simulink model "alveo_onehundred_gbe"  (R2021a)
settings: Solver=VariableStepAuto  StartTime=0.0  StopTime=10.0  RelTol=1e-3
libraries: xbsIndex_r4 x30
settings Model: Creator=qwerty40  LastModifiedBy=wnew
settings SolverCC: AlgebraicLoopSolver=TrustRegion
settings DataIOCC: ReturnWorkspaceOutputs=off
settings DebuggingCC: SFMachineParentedDataDiag=warning  ArithmeticOperatorsInVariantConditions=warning
settings SFSimCC: SimUseLocalCustomCode=off  CustomCodeUndefinedFunction=UseInterfaceOnly
settings RTWCC: RTWUseLocalCustomCode=off
settings CodeAppCC: StateflowObjectComments=on

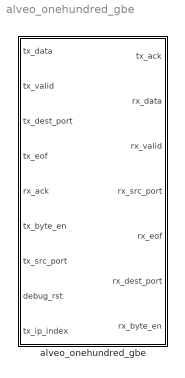
== system alveo_onehundred_gbe ==
  alveo_onehundred_gbe : Subsystem  Tag=xps:onehundred_gbe  mask(alveo_onehundred_gbe){Parameter1=off, fab_mac=hex2dec('123456780000'), fab_ip=192*(2^24) + 168*(2^16) + 5*(2^8) + 20*(2^0), fab_udp=10000}
      mask prompts: Parameter1 "Farm Mode"; fab_mac "Fabric MAC Address"; fab_ip "Fabric IP Address"; fab_udp "Fabric UDP Port"
      mask help: This block sends and receives UDP frames (packets). It accepts a 64 bit wide data stream with user-determined frame breaks. The data stream is wrapped in a UDP frame for transmission. Incoming UDP packets are unwrapped and the data presented as a 64 bit wide stream.
      mask init:
      | alveo_onehundred_gbe_mask(gcb)
      settings: AttributesFormatString=incoming_latency=0

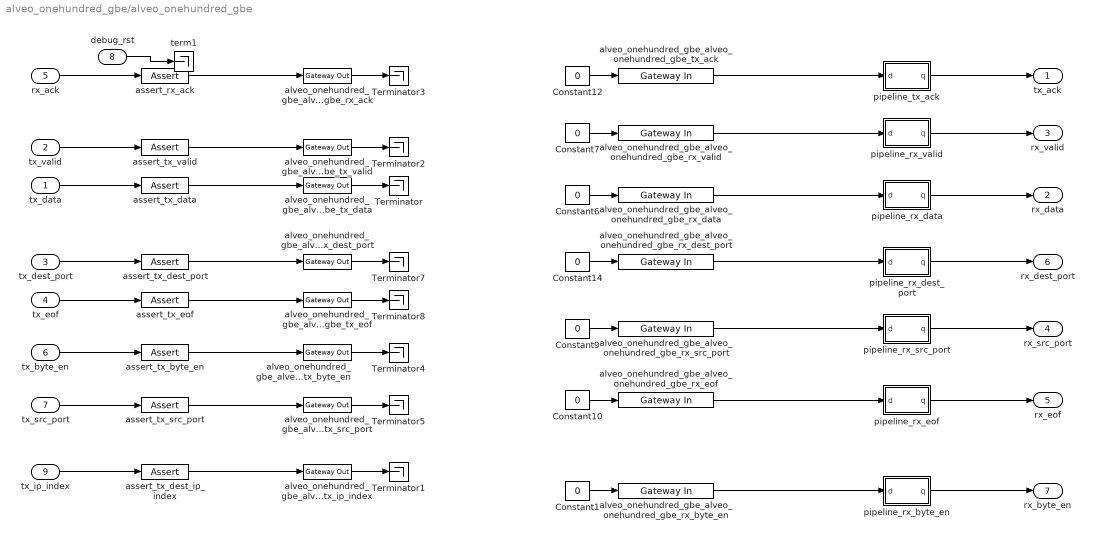
== system alveo_onehundred_gbe/alveo_onehundred_gbe ==
  tx_data : Inport
  tx_valid : Inport  Port=2
  tx_dest_port : Inport  Port=3
  tx_eof : Inport  Port=4
  rx_ack : Inport  Port=5
  tx_byte_en : Inport  Port=6
  tx_src_port : Inport  Port=7
  debug_rst : Inport  Port=8
  tx_ip_index : Inport  Port=9
  Constant{1,6..7,9..10,12,14} (7 alike) : Constant  Value=0
  Terminator{,1..5,7..8} (8 alike) : Terminator
  alveo_onehundred_gbe_alveo_onehundred_gbe_rx_ack : xbsIndex_r4/Gateway Out  inherit_from_input=off  hdl_port=on  rows=1  columns=1  UseAsDAC=off  DACChannel='1'  interface=None  automatic_assignment=on  address_offset=hex2dec('00')  intf_name=''  intf_description=''  timing_constraint=None  locs_specified=off  LOCs={}  io_standard={}  block_type=gatewayout
      settings: infoedit="Gateway out block.  Converts Xilinx fixed point inputs into ouputs of type Simulink integer, double, or fixed point.<P><P>Hardware notes:  In hardware these blocks become top level output ports or are discarded, depending on how they are configured."  xl_area=[0, 0, 0, 0, 0, 0, 0]
  alveo_onehundred_gbe_alveo_onehundred_gbe_rx_byte_en : xbsIndex_r4/Gateway In  gui_display_data_type=Fixed-point  arith_type=Unsigned  n_bits=64  bin_pt=0  preci_type=Single  exp_width=8  frac_width=24  rows=1  columns=1  quantization=Truncate  overflow=Wrap  period=1  UseAsADC=off  ADCChannel='1'  interface=None  automatic_assignment=on  address_offset=hex2dec('00')  intf_name=''  intf_description=''  default_value=0  timing_constraint=None  locs_specified=off  LOCs={}  io_standard={}  inherit_from_input=off  hdl_port=on  dbl_ovrd=off  block_type=gatewayin
      settings: xl_area=[0, 0, 0, 0, 0, 0, 0]
  alveo_onehundred_gbe_alveo_onehundred_gbe_rx_data : xbsIndex_r4/Gateway In  gui_display_data_type=Fixed-point  arith_type=Unsigned  n_bits=512  bin_pt=0  preci_type=Single  exp_width=8  frac_width=24  rows=1  columns=1  quantization=Truncate  overflow=Wrap  period=1  UseAsADC=off  ADCChannel='1'  interface=None  automatic_assignment=on  address_offset=hex2dec('00')  intf_name=''  intf_description=''  default_value=0  timing_constraint=None  locs_specified=off  LOCs={}  io_standard={}  inherit_from_input=off  hdl_port=on  dbl_ovrd=off  block_type=gatewayin
      settings: xl_area=[0, 0, 0, 0, 0, 0, 0]
  alveo_onehundred_gbe_alveo_onehundred_gbe_rx_dest_port : xbsIndex_r4/Gateway In  gui_display_data_type=Fixed-point  arith_type=Unsigned  n_bits=16  bin_pt=0  preci_type=Single  exp_width=8  frac_width=24  rows=1  columns=1  quantization=Truncate  overflow=Wrap  period=1  UseAsADC=off  ADCChannel='1'  interface=None  automatic_assignment=on  address_offset=hex2dec('00')  intf_name=''  intf_description=''  default_value=0  timing_constraint=None  locs_specified=off  LOCs={}  io_standard={}  inherit_from_input=off  hdl_port=on  dbl_ovrd=off  block_type=gatewayin
      settings: infoedit="Gateway in block.  Converts inputs of type Simulink integer, double and fixed point to  Xilinx fixed point type.<P><P>Hardware notes:  In hardware these blocks become top level input ports."  xl_area=[0, 0, 0, 0, 0, 0, 0]
  alveo_onehundred_gbe_alveo_onehundred_gbe_rx_eof : xbsIndex_r4/Gateway In  gui_display_data_type=Fixed-point  arith_type=Boolean  n_bits=1  bin_pt=0  preci_type=Single  exp_width=8  frac_width=24  rows=1  columns=1  quantization=Truncate  overflow=Wrap  period=1  UseAsADC=off  ADCChannel='1'  interface=None  automatic_assignment=on  address_offset=hex2dec('00')  intf_name=''  intf_description=''  default_value=0  timing_constraint=None  locs_specified=off  LOCs={}  io_standard={}  inherit_from_input=off  hdl_port=on  dbl_ovrd=off  block_type=gatewayin
      settings: infoedit="Gateway in block.  Converts inputs of type Simulink integer, double and fixed point to  Xilinx fixed point type.<P><P>Hardware notes:  In hardware these blocks become top level input ports."  xl_area=[0, 0, 0, 0, 0, 0, 0]
  alveo_onehundred_gbe_alveo_onehundred_gbe_rx_src_port : xbsIndex_r4/Gateway In  gui_display_data_type=Fixed-point  arith_type=Unsigned  n_bits=16  bin_pt=0  preci_type=Single  exp_width=8  frac_width=24  rows=1  columns=1  quantization=Truncate  overflow=Wrap  period=1  UseAsADC=off  ADCChannel='1'  interface=None  automatic_assignment=on  address_offset=hex2dec('00')  intf_name=''  intf_description=''  default_value=0  timing_constraint=None  locs_specified=off  LOCs={}  io_standard={}  inherit_from_input=off  hdl_port=on  dbl_ovrd=off  block_type=gatewayin
      settings: infoedit="Gateway in block.  Converts inputs of type Simulink integer, double and fixed point to  Xilinx fixed point type.<P><P>Hardware notes:  In hardware these blocks become top level input ports."  xl_area=[0, 0, 0, 0, 0, 0, 0]
  alveo_onehundred_gbe_alveo_onehundred_gbe_rx_valid : xbsIndex_r4/Gateway In  gui_display_data_type=Boolean  arith_type=Boolean  n_bits=4  bin_pt=0  preci_type=Single  exp_width=8  frac_width=24  rows=1  columns=1  quantization=Truncate  overflow=Wrap  period=1  UseAsADC=off  ADCChannel='1'  interface=None  automatic_assignment=on  address_offset=hex2dec('00')  intf_name=''  intf_description=''  default_value=0  timing_constraint=None  locs_specified=off  LOCs={}  io_standard={}  inherit_from_input=off  hdl_port=on  dbl_ovrd=off  block_type=gatewayin
      settings: xl_area=[0, 0, 0, 0, 0, 0, 0]
  alveo_onehundred_gbe_alveo_onehundred_gbe_tx_ack : xbsIndex_r4/Gateway In  gui_display_data_type=Boolean  arith_type=Boolean  n_bits=1  bin_pt=0  preci_type=Single  exp_width=8  frac_width=24  rows=1  columns=1  quantization=Truncate  overflow=Wrap  period=1  UseAsADC=off  ADCChannel='1'  interface=None  automatic_assignment=on  address_offset=hex2dec('00')  intf_name=''  intf_description=''  default_value=0  timing_constraint=None  locs_specified=off  LOCs={}  io_standard={}  inherit_from_input=off  hdl_port=on  dbl_ovrd=off  block_type=gatewayin
      settings: xl_area=[0, 0, 0, 0, 0, 0, 0]
  alveo_onehundred_gbe_alveo_onehundred_gbe_tx_byte_en : xbsIndex_r4/Gateway Out  inherit_from_input=off  hdl_port=on  rows=1  columns=1  UseAsDAC=off  DACChannel='1'  interface=None  automatic_assignment=on  address_offset=hex2dec('00')  intf_name=''  intf_description=''  timing_constraint=None  locs_specified=off  LOCs={}  io_standard={}  block_type=gatewayout
      settings: xl_area=[0, 0, 0, 0, 0, 0, 0]
  alveo_onehundred_gbe_alveo_onehundred_gbe_tx_data : xbsIndex_r4/Gateway Out  inherit_from_input=off  hdl_port=on  rows=1  columns=1  UseAsDAC=off  DACChannel='1'  interface=None  automatic_assignment=on  address_offset=hex2dec('00')  intf_name=''  intf_description=''  timing_constraint=None  locs_specified=off  LOCs={}  io_standard={}  block_type=gatewayout
      settings: infoedit="Gateway out block.  Converts Xilinx fixed point inputs into ouputs of type Simulink integer, double, or fixed point.<P><P>Hardware notes:  In hardware these blocks become top level output ports or are discarded, depending on how they are configured."  xl_area=[0, 0, 0, 0, 0, 0, 0]
  alveo_onehundred_gbe_alveo_onehundred_gbe_tx_dest_port : xbsIndex_r4/Gateway Out  inherit_from_input=off  hdl_port=on  rows=1  columns=1  UseAsDAC=off  DACChannel='1'  interface=None  automatic_assignment=on  address_offset=hex2dec('00')  intf_name=''  intf_description=''  timing_constraint=None  locs_specified=off  LOCs={}  io_standard={}  block_type=gatewayout
      settings: infoedit="Gateway out block.  Converts Xilinx fixed point inputs into ouputs of type Simulink integer, double, or fixed point.<P><P>Hardware notes:  In hardware these blocks become top level output ports or are discarded, depending on how they are configured."  xl_area=[0, 0, 0, 0, 0, 0, 0]
  alveo_onehundred_gbe_alveo_onehundred_gbe_tx_eof : xbsIndex_r4/Gateway Out  inherit_from_input=off  hdl_port=on  rows=1  columns=1  UseAsDAC=off  DACChannel='1'  interface=None  automatic_assignment=on  address_offset=hex2dec('00')  intf_name=''  intf_description=''  timing_constraint=None  locs_specified=off  LOCs={}  io_standard={}  block_type=gatewayout
      settings: infoedit="Gateway out block.  Converts Xilinx fixed point inputs into ouputs of type Simulink integer, double, or fixed point.<P><P>Hardware notes:  In hardware these blocks become top level output ports or are discarded, depending on how they are configured."  xl_area=[0, 0, 0, 0, 0, 0, 0]
  alveo_onehundred_gbe_alveo_onehundred_gbe_tx_ip_index : xbsIndex_r4/Gateway Out  inherit_from_input=off  hdl_port=on  rows=1  columns=1  UseAsDAC=off  DACChannel='1'  interface=None  automatic_assignment=on  address_offset=hex2dec('00')  intf_name=''  intf_description=''  timing_constraint=None  locs_specified=off  LOCs={}  io_standard={}  block_type=gatewayout
      settings: infoedit="Gateway out block.  Converts Xilinx fixed point inputs into ouputs of type Simulink integer, double, or fixed point.<P><P>Hardware notes:  In hardware these blocks become top level output ports or are discarded, depending on how they are configured."  xl_area=[0, 0, 0, 0, 0, 0, 0]
  alveo_onehundred_gbe_alveo_onehundred_gbe_tx_src_port : xbsIndex_r4/Gateway Out  inherit_from_input=off  hdl_port=on  rows=1  columns=1  UseAsDAC=off  DACChannel='1'  interface=None  automatic_assignment=on  address_offset=hex2dec('00')  intf_name=''  intf_description=''  timing_constraint=None  locs_specified=off  LOCs={}  io_standard={}  block_type=gatewayout
      settings: infoedit="Gateway out block.  Converts Xilinx fixed point inputs into ouputs of type Simulink integer, double, or fixed point.<P><P>Hardware notes:  In hardware these blocks become top level output ports or are discarded, depending on how they are configured."  xl_area=[0, 0, 0, 0, 0, 0, 0]
  alveo_onehundred_gbe_alveo_onehundred_gbe_tx_valid : xbsIndex_r4/Gateway Out  inherit_from_input=off  hdl_port=on  rows=1  columns=1  UseAsDAC=off  DACChannel='1'  interface=None  automatic_assignment=on  address_offset=hex2dec('00')  intf_name=''  intf_description=''  timing_constraint=None  locs_specified=off  LOCs={}  io_standard={}  block_type=gatewayout
      settings: infoedit="Gateway out block.  Converts Xilinx fixed point inputs into ouputs of type Simulink integer, double, or fixed point.<P><P>Hardware notes:  In hardware these blocks become top level output ports or are discarded, depending on how they are configured."  xl_area=[0, 0, 0, 0, 0, 0, 0]
  assert_rx_ack : xbsIndex_r4/Assert  assert_type=on  type_source=Explicitly  gui_display_data_type=Boolean  arith_type=Boolean  n_bits=16  bin_pt=0  preci_type=Single  exp_width=8  frac_width=24  assert_rate=on  rate_source=Explicitly  period=1  output_port=on  block_type=assert
  assert_tx_byte_en : xbsIndex_r4/Assert  assert_type=on  type_source=Explicitly  gui_display_data_type=Fixed-point  arith_type=Unsigned  n_bits=64  bin_pt=0  preci_type=Single  exp_width=8  frac_width=24  assert_rate=on  rate_source=Explicitly  period=1  output_port=on  block_type=assert
  assert_tx_data : xbsIndex_r4/Assert  assert_type=on  type_source=Explicitly  gui_display_data_type=Fixed-point  arith_type=Unsigned  n_bits=512  bin_pt=0  preci_type=Single  exp_width=8  frac_width=24  assert_rate=on  rate_source=Explicitly  period=1  output_port=on  block_type=assert
  assert_tx_dest_ip_index : xbsIndex_r4/Assert  assert_type=on  type_source=Explicitly  gui_display_data_type=Fixed-point  arith_type=Unsigned  n_bits=8  bin_pt=0  preci_type=Single  exp_width=8  frac_width=24  assert_rate=on  rate_source=Explicitly  period=1  output_port=on  block_type=assert
  assert_tx_dest_port : xbsIndex_r4/Assert  assert_type=on  type_source=Explicitly  gui_display_data_type=Fixed-point  arith_type=Unsigned  n_bits=16  bin_pt=0  preci_type=Single  exp_width=8  frac_width=24  assert_rate=on  rate_source=Explicitly  period=1  output_port=on  block_type=assert
  assert_tx_eof : xbsIndex_r4/Assert  assert_type=on  type_source=Explicitly  gui_display_data_type=Boolean  arith_type=Boolean  n_bits=16  bin_pt=0  preci_type=Single  exp_width=8  frac_width=24  assert_rate=on  rate_source=Explicitly  period=1  output_port=on  block_type=assert
  assert_tx_src_port : xbsIndex_r4/Assert  assert_type=on  type_source=Explicitly  gui_display_data_type=Fixed-point  arith_type=Unsigned  n_bits=16  bin_pt=0  preci_type=Single  exp_width=8  frac_width=24  assert_rate=on  rate_source=Explicitly  period=1  output_port=on  block_type=assert
  assert_tx_valid : xbsIndex_r4/Assert  assert_type=on  type_source=Explicitly  gui_display_data_type=Boolean  arith_type=Boolean  n_bits=16  bin_pt=14  preci_type=Single  exp_width=8  frac_width=24  assert_rate=on  rate_source=Explicitly  period=1  output_port=on  block_type=assert
  pipeline_rx_byte_en : Subsystem  AncestorBlock=casper_library_delays/pipeline  mask(pipeline){csp_latency=1}
      mask prompts: csp_latency "Latency"
      mask help:
      | An explicitly laid-out delay line to avoid mapping to SRL16s
      | for use in pipelining to help achieve timing closure.
      mask init:
      | pipeline_init(gcb,'latency',csp_latency);
      settings: AttributesFormatString=Latency = %<latency>
      mask Display:
      | port_label('input', 1, 'd');
      | port_label('output', 1, 'q');
      | disp(['Z^-', num2str(csp_latency)]);
  pipeline_rx_data : Subsystem  AncestorBlock=casper_library_delays/pipeline  mask(pipeline){csp_latency=1}
      mask prompts: csp_latency "Latency"
      mask help:
      | An explicitly laid-out delay line to avoid mapping to SRL16s
      | for use in pipelining to help achieve timing closure.
      mask init:
      | pipeline_init(gcb,'latency',csp_latency);
      settings: AttributesFormatString=Latency = %<latency>
      mask Display:
      | port_label('input', 1, 'd');
      | port_label('output', 1, 'q');
      | disp(['Z^-', num2str(csp_latency)]);
  pipeline_rx_dest_port : Subsystem  AncestorBlock=casper_library_delays/pipeline  mask(pipeline){csp_latency=1}
      mask prompts: csp_latency "Latency"
      mask help:
      | An explicitly laid-out delay line to avoid mapping to SRL16s
      | for use in pipelining to help achieve timing closure.
      mask init:
      | pipeline_init(gcb,'latency',csp_latency);
      settings: AttributesFormatString=Latency = %<latency>
      mask Display:
      | port_label('input', 1, 'd');
      | port_label('output', 1, 'q');
      | disp(['Z^-', num2str(csp_latency)]);
  pipeline_rx_eof : Subsystem  AncestorBlock=casper_library_delays/pipeline  mask(pipeline){csp_latency=1}
      mask prompts: csp_latency "Latency"
      mask help:
      | An explicitly laid-out delay line to avoid mapping to SRL16s
      | for use in pipelining to help achieve timing closure.
      mask init:
      | pipeline_init(gcb,'latency',csp_latency);
      settings: AttributesFormatString=Latency = %<latency>
      mask Display:
      | port_label('input', 1, 'd');
      | port_label('output', 1, 'q');
      | disp(['Z^-', num2str(csp_latency)]);
  pipeline_rx_src_port : Subsystem  AncestorBlock=casper_library_delays/pipeline  mask(pipeline){csp_latency=1}
      mask prompts: csp_latency "Latency"
      mask help:
      | An explicitly laid-out delay line to avoid mapping to SRL16s
      | for use in pipelining to help achieve timing closure.
      mask init:
      | pipeline_init(gcb,'latency',csp_latency);
      settings: AttributesFormatString=Latency = %<latency>
      mask Display:
      | port_label('input', 1, 'd');
      | port_label('output', 1, 'q');
      | disp(['Z^-', num2str(csp_latency)]);
  pipeline_rx_valid : Subsystem  AncestorBlock=casper_library_delays/pipeline  mask(pipeline){csp_latency=1}
      mask prompts: csp_latency "Latency"
      mask help:
      | An explicitly laid-out delay line to avoid mapping to SRL16s
      | for use in pipelining to help achieve timing closure.
      mask init:
      | pipeline_init(gcb,'latency',csp_latency);
      settings: AttributesFormatString=Latency = %<latency>
      mask Display:
      | port_label('input', 1, 'd');
      | port_label('output', 1, 'q');
      | disp(['Z^-', num2str(csp_latency)]);
  pipeline_tx_ack : Subsystem  AncestorBlock=casper_library_delays/pipeline  mask(pipeline){csp_latency=1}
      mask prompts: csp_latency "Latency"
      mask help:
      | An explicitly laid-out delay line to avoid mapping to SRL16s
      | for use in pipelining to help achieve timing closure.
      mask init:
      | pipeline_init(gcb,'latency',csp_latency);
      settings: AttributesFormatString=Latency = %<latency>
      mask Display:
      | port_label('input', 1, 'd');
      | port_label('output', 1, 'q');
      | disp(['Z^-', num2str(csp_latency)]);
  term1 : Terminator
  tx_ack : Outport  VectorParamsAs1DForOutWhenUnconnected=off
  rx_data : Outport  Port=2  VectorParamsAs1DForOutWhenUnconnected=off
  rx_valid : Outport  Port=3  VectorParamsAs1DForOutWhenUnconnected=off
  rx_src_port : Outport  Port=4  VectorParamsAs1DForOutWhenUnconnected=off
  rx_eof : Outport  Port=5  VectorParamsAs1DForOutWhenUnconnected=off
  rx_dest_port : Outport  Port=6  VectorParamsAs1DForOutWhenUnconnected=off
  rx_byte_en : Outport  Port=7  VectorParamsAs1DForOutWhenUnconnected=off
  wires:
  tx_valid/1 -> assert_tx_valid/1
  pipeline_rx_eof/1(q) -> rx_eof/1
  pipeline_rx_dest_port/1(q) -> rx_dest_port/1
  pipeline_rx_src_port/1(q) -> rx_src_port/1
  Constant14/1 -> alveo_onehundred_gbe_alveo_onehundred_gbe_rx_dest_port/1
  alveo_onehundred_gbe_alveo_onehundred_gbe_rx_dest_port/1 -> pipeline_rx_dest_port/1(d)
  alveo_onehundred_gbe_alveo_onehundred_gbe_tx_ack/1 -> pipeline_tx_ack/1(d)
  Constant12/1 -> alveo_onehundred_gbe_alveo_onehundred_gbe_tx_ack/1
  rx_ack/1 -> assert_rx_ack/1
  assert_rx_ack/1 -> alveo_onehundred_gbe_alveo_onehundred_gbe_rx_ack/1
  alveo_onehundred_gbe_alveo_onehundred_gbe_rx_data/1 -> pipeline_rx_data/1(d)
  tx_data/1 -> assert_tx_data/1
  assert_tx_data/1 -> alveo_onehundred_gbe_alveo_onehundred_gbe_tx_data/1
  assert_tx_valid/1 -> alveo_onehundred_gbe_alveo_onehundred_gbe_tx_valid/1
  alveo_onehundred_gbe_alveo_onehundred_gbe_tx_data/1 -> Terminator/1
  alveo_onehundred_gbe_alveo_onehundred_gbe_tx_valid/1 -> Terminator2/1
  Constant6/1 -> alveo_onehundred_gbe_alveo_onehundred_gbe_rx_data/1
  alveo_onehundred_gbe_alveo_onehundred_gbe_rx_ack/1 -> Terminator3/1
  Constant7/1 -> alveo_onehundred_gbe_alveo_onehundred_gbe_rx_valid/1
  tx_dest_port/1 -> assert_tx_dest_port/1
  assert_tx_dest_port/1 -> alveo_onehundred_gbe_alveo_onehundred_gbe_tx_dest_port/1
  alveo_onehundred_gbe_alveo_onehundred_gbe_tx_dest_port/1 -> Terminator7/1
  tx_eof/1 -> assert_tx_eof/1
  assert_tx_eof/1 -> alveo_onehundred_gbe_alveo_onehundred_gbe_tx_eof/1
  alveo_onehundred_gbe_alveo_onehundred_gbe_tx_eof/1 -> Terminator8/1
  Constant9/1 -> alveo_onehundred_gbe_alveo_onehundred_gbe_rx_src_port/1
  alveo_onehundred_gbe_alveo_onehundred_gbe_rx_src_port/1 -> pipeline_rx_src_port/1(d)
  Constant10/1 -> alveo_onehundred_gbe_alveo_onehundred_gbe_rx_eof/1
  alveo_onehundred_gbe_alveo_onehundred_gbe_rx_eof/1 -> pipeline_rx_eof/1(d)
  alveo_onehundred_gbe_alveo_onehundred_gbe_rx_valid/1 -> pipeline_rx_valid/1(d)
  pipeline_rx_valid/1(q) -> rx_valid/1
  pipeline_tx_ack/1(q) -> tx_ack/1
  pipeline_rx_data/1(q) -> rx_data/1
  ? -> ?
  ? -> ?
  alveo_onehundred_gbe_alveo_onehundred_gbe_tx_byte_en/1 -> Terminator4/1
  assert_tx_byte_en/1 -> alveo_onehundred_gbe_alveo_onehundred_gbe_tx_byte_en/1
  tx_byte_en/1 -> assert_tx_byte_en/1
  pipeline_rx_byte_en/1(q) -> rx_byte_en/1
  alveo_onehundred_gbe_alveo_onehundred_gbe_rx_byte_en/1 -> pipeline_rx_byte_en/1(d)
  Constant1/1 -> alveo_onehundred_gbe_alveo_onehundred_gbe_rx_byte_en/1
  tx_src_port/1 -> assert_tx_src_port/1
  alveo_onehundred_gbe_alveo_onehundred_gbe_tx_src_port/1 -> Terminator5/1
  assert_tx_src_port/1 -> alveo_onehundred_gbe_alveo_onehundred_gbe_tx_src_port/1
  debug_rst/1 -> term1/1
  alveo_onehundred_gbe_alveo_onehundred_gbe_tx_ip_index/1 -> Terminator1/1
  assert_tx_dest_ip_index/1 -> alveo_onehundred_gbe_alveo_onehundred_gbe_tx_ip_index/1
  tx_ip_index/1 -> assert_tx_dest_ip_index/1

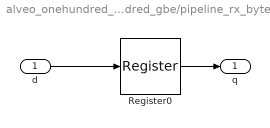
== system alveo_onehundred_gbe/alveo_onehundred_gbe/pipeline_rx_byte_en ==
  d : Inport
  Register0 : xbsIndex_r4/Register  init=0  rst=off  en=off  dbl_ovrd=off  block_type=register
  q : Outport  VectorParamsAs1DForOutWhenUnconnected=off
  wires:
  d/1 -> Register0/1
  Register0/1 -> q/1

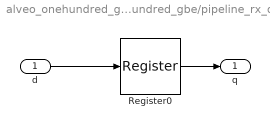
== system alveo_onehundred_gbe/alveo_onehundred_gbe/pipeline_rx_data ==
  d : Inport
  Register0 : xbsIndex_r4/Register  init=0  rst=off  en=off  dbl_ovrd=off  block_type=register
  q : Outport  VectorParamsAs1DForOutWhenUnconnected=off
  wires:
  d/1 -> Register0/1
  Register0/1 -> q/1

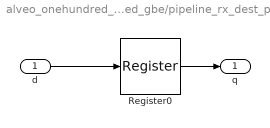
== system alveo_onehundred_gbe/alveo_onehundred_gbe/pipeline_rx_dest_port ==
  d : Inport
  Register0 : xbsIndex_r4/Register  init=0  rst=off  en=off  dbl_ovrd=off  block_type=register
  q : Outport  VectorParamsAs1DForOutWhenUnconnected=off
  wires:
  d/1 -> Register0/1
  Register0/1 -> q/1

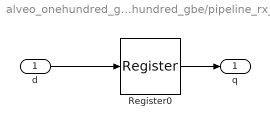
== system alveo_onehundred_gbe/alveo_onehundred_gbe/pipeline_rx_eof ==
  d : Inport
  Register0 : xbsIndex_r4/Register  init=0  rst=off  en=off  dbl_ovrd=off  block_type=register
  q : Outport  VectorParamsAs1DForOutWhenUnconnected=off
  wires:
  d/1 -> Register0/1
  Register0/1 -> q/1

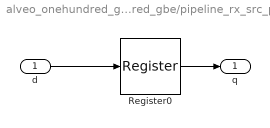
== system alveo_onehundred_gbe/alveo_onehundred_gbe/pipeline_rx_src_port ==
  d : Inport
  Register0 : xbsIndex_r4/Register  init=0  rst=off  en=off  dbl_ovrd=off  block_type=register
  q : Outport  VectorParamsAs1DForOutWhenUnconnected=off
  wires:
  d/1 -> Register0/1
  Register0/1 -> q/1

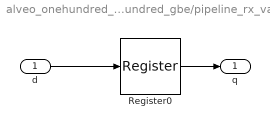
== system alveo_onehundred_gbe/alveo_onehundred_gbe/pipeline_rx_valid ==
  d : Inport
  Register0 : xbsIndex_r4/Register  init=0  rst=off  en=off  dbl_ovrd=off  block_type=register
  q : Outport  VectorParamsAs1DForOutWhenUnconnected=off
  wires:
  d/1 -> Register0/1
  Register0/1 -> q/1

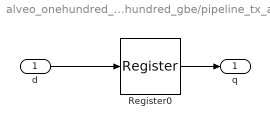
== system alveo_onehundred_gbe/alveo_onehundred_gbe/pipeline_tx_ack ==
  d : Inport
  Register0 : xbsIndex_r4/Register  init=0  rst=off  en=off  dbl_ovrd=off  block_type=register
  q : Outport  VectorParamsAs1DForOutWhenUnconnected=off
  wires:
  d/1 -> Register0/1
  Register0/1 -> q/1
